simulink library "WECSim_Lib_Cables"  (R2020b)
settings: Solver=VariableStepAuto  StartTime=0.0  StopTime=10.0  RelTol=1e-3
undefined symbols (not defined in the file or in its folder): cable, simu, X, Y, Z
libraries: sm_lib x15, nesl_utility x13, vrlib x2, WECSim_Lib_Body_Elements x2
settings Model: Creator=kmruehl  LastModifiedBy=akeeste

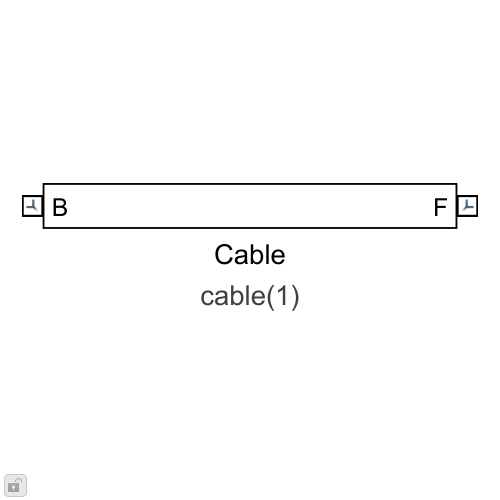
[thumbnail: Simulink's stored preview of the top-level diagram]
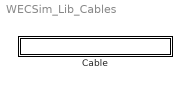
== system WECSim_Lib_Cables ==
  Cable : Subsystem  VariantControl=sv_Cable3DOF  mask(Cables){cable=cable(1)}
      mask prompts: cable "Cable Name:"
      mask help:
      | A cable that can be used to connect two bodies. If connecting a body to the seabed, use "Mooring" instead. This cable attaches to the body at either end with a spherical joint and applies damping and spring force between the bodies if the cable is in tension, and no force otherwise.
      |
      | The variable name input below must be 'cable(i)' where i=1,2,...
      | cable(i) must be defined in the input file with the following fields:
      |
      |   .name (required)
      | 	String.
      | 	Constraint name. Must comply with Matlab's variable naming rules.
      |   .stiffness (required)
      | 	The spring stiffness of the cable, applied externally as an actuation to the
      | 	translational PTO. This should be a strictly positive value for the cable to
      | 	act in tension. Default = 0
      |   .damping (required)
      | 	The damping coefficient of the cable, applied externally as an actuation to the
      | 	translational PTO. This should be a strictly positive value for the cable to
      | 	act in tension. Default = 0
      |   .length (optional)
      | 	The equilibrium length of the cable. If unspecified, it will be set at equilibrium
      | 	initially.
      |   .base.location (required)
      | 	The location of the top spherical joint connecting the cable to block base.
      | 	Default = [999 999 999]
      |   .follower.location (required)
      | 	The location of the bottom spherical joint connecting the cable to block follower.
      | 	Default = [999 999 999]
      mask init:
      | % toWorkspace
      | h=[gcb '/To Workspace'];
      | responseName=['cable' num2str((cable.number)) '_out'];
      | set_param(h,'VariableName',responseName);
      | 
      | %% follower drag body
      | % bodyMass constant
      | h=[gcb '/Follower Drag Body/Body Mass']; 
      | set_param(h,'Value', num2str(cable.mass));
      | % velocity GoTo
      | h=[gcb '/Follower Drag Body/Goto1'];
      | responseName=['cableVel' num2str((cable.number)) '_out1'];
      | set_param(h,'GotoTag',responseName);
      | % velocity From
      | h=[gcb '/Follower Drag Body/From1'];
      | responseName=['cableVel' num2str((cable.number)) '_out1'];
      | set_param(h,'GotoTag',responseName);
      | 
      | %% base drag body
      | % bodyMass constant
      | h=[gcb '/Base Drag Body/Body Mass']; 
      | set_param(h,'Value', num2str(cable.mass));
      | % velocity GoTo
      | h=[gcb '/Base Drag Body/Goto1'];
      | responseName=['cableVel' num2str((cable.number)) '_out2'];
      | set_param(h,'GotoTag',responseName);
      | % velocity From
      | h=[gcb '/Base Drag Body/From1'];
      | responseName=['cableVel' num2str((cable.number)) '_out2'];
      | set_param(h,'GotoTag',responseName);
      settings: AttributesFormatString=%<cable>
      mask Help:
      | A cable that can be used to connect two bodies. If connecting a body to the seabed, use "Mooring" instead. This cable attaches to the body at either end with a spherical joint and applies damping and spring force between the bodies if the cable is in tension, and no force otherwise.
      | 
      | The variable name input below must be 'cable(i)' where i=1,2,...
      | cable(i) must be defined in the input file with the following fields:
      | 
      |   .name (required)
      | 	String.
      | 	Constraint name. Must comply with Matlab's variable naming rules.
      |   .stiffness (required)
      | 	The spring stiffness of the cable, applied externally as an actuation to the
      | 	translational PTO. This should be a strictly positive value for the cable to
      | 	act in tension. Default = 0
      |   .damping (required)
      | 	The damping coefficient of the cable, applied externally as an actuation to the
      | 	translational PTO. This should be a strictly positive value for the cable to
      | 	act in tension. Default = 0
      |   .length (optional)
      | 	The equilibrium length of the cable. If unspecified, it will be set at equilibrium
      | 	initially.
      |   .base.location (required)
      | 	The location of the top spherical joint connecting the cable to block base.
      | 	Default = [999 999 999]
      |   .follower.location (required)
      | 	The location of the bottom spherical joint connecting the cable to block follower.
      | 	Default = [999 999 999]

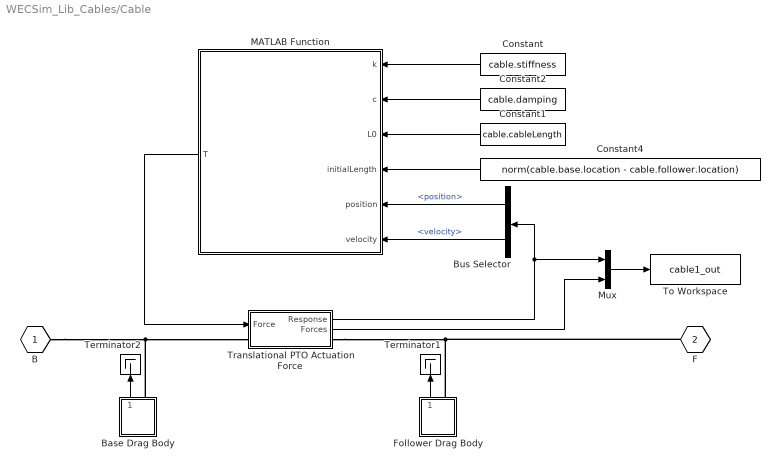
== system WECSim_Lib_Cables/Cable ==
  Base Drag Body : Subsystem  VariantControl=sv_b1_dragBody  mask(Drag Body){}
      mask help:
      | A drag body contains six degrees of freedom in x, y, z and Mx, My, Mz. It contains a buoyant force, linear damping force, and Morison Element and viscous forces. It is not influenced by wave excitation, radiation damping or radiation added mass.
      |
      | The variable name input below must be 'body(i)' where i=1,2,...
      | body(i) must be defined in the input file with the following fields:
      |
      |     .mass (required)
      |             Float or string.
      |             The translational interia or mass of the body in kg. If a string, the value must be 'equilibrium'. Default = [ ]
      |     .momOfIntertia (required)
      |             3x1 vector [Ixx Iyy Izz].
      |             Rotational intertia of the body in kg*m^2. Default = [ ]
      |     .filename (required)
      |             String.
      |             The file path specifying the .h5 file for the body.
      |     .name (optional)
      |             String.
      |             Specifies the body name. Default = [ ]
      |     .cg (optional)
      |             3x1 float vector [x y z]
      |     .cb (optional)
      |             3x1 float vector [x y z]
      |             Body center of buoyancy in m. Default = [ ].
      |     .volume (optional)
      |             Float.
      |             Displaced volume at the equilibrium position in m^3. Default = [ ]
      |     .geometryFile (optional)
      |             String
      |             Path to the geometry file of the body (.stl). Required for nonlinear hydrodynamics or visualization. Default = [ ]
  Bus Selector : BusSelector  OutputSignals=position,velocity
  Constant : Constant  Value=cable.stiffness
  Constant1 : Constant  Value=cable.cableLength
  Constant2 : Constant  Value=cable.damping
  Constant4 : Constant  Value=norm(cable.base.location - cable.follower.location)
  Follower Drag Body : Subsystem  VariantControl=sv_b1_dragBody  mask(Drag Body){}
      mask help:
      | A drag body contains six degrees of freedom in x, y, z and Mx, My, Mz. It contains a buoyant force, linear damping force, and Morison Element and viscous forces. It is not influenced by wave excitation, radiation damping or radiation added mass.
      |
      | The variable name input below must be 'body(i)' where i=1,2,...
      | body(i) must be defined in the input file with the following fields:
      |
      |     .mass (required)
      |             Float or string.
      |             The translational interia or mass of the body in kg. If a string, the value must be 'equilibrium'. Default = [ ]
      |     .momOfIntertia (required)
      |             3x1 vector [Ixx Iyy Izz].
      |             Rotational intertia of the body in kg*m^2. Default = [ ]
      |     .filename (required)
      |             String.
      |             The file path specifying the .h5 file for the body.
      |     .name (optional)
      |             String.
      |             Specifies the body name. Default = [ ]
      |     .cg (optional)
      |             3x1 float vector [x y z]
      |     .cb (optional)
      |             3x1 float vector [x y z]
      |             Body center of buoyancy in m. Default = [ ].
      |     .volume (optional)
      |             Float.
      |             Displaced volume at the equilibrium position in m^3. Default = [ ]
      |     .geometryFile (optional)
      |             String
      |             Path to the geometry file of the body (.stl). Required for nonlinear hydrodynamics or visualization. Default = [ ]
  MATLAB Function : MATLAB Function  TreatAsAtomicUnit=on
  Mux : Mux  Inputs=2
  Terminator1 : Terminator
  Terminator2 : Terminator
  To Workspace : ToWorkspace  VariableName=cable1_out  SaveFormat=Structure With Time  SampleTime=simu.dtOut
  Translational PTO Actuation Force : Subsystem  mask(PTO){cable=cable}
      mask help:
      | Constrains the follower to translational motion relative to the base, in
      | the PTO's Z-direction and adds PTO stiffness and damping. Also applies a
      | user-defined force and outputs extension, velocity, and acceleration.
      |
      |
      | The variable name input below must be 'pto(i)' where i=1,2,...
      | pto(i) must be defined in the input file with the following fields:
      |
      |     .name (required)
      |             String.
      |             PTO name. Must comply with Matlab's variable naming rules.
      |     .loc (optional)
      |             3x1 vector [x y z] in meters.
      |             PTO location. Default = [0 0 0]
      |     .k (optional)
      |             Float.
      |             PTO linear spring stiffness. Default = 0
      |     .c (optional)
      |             Float.
      |             PTO linear damping coefficient. Default = 0
      |     .orientation.z (optional)
      |             3x1 vector [x y z].
      |             Direction of the PTO's Z-coordinate. Default = [0 0 1]
      |     .orientation.y (optional)
      |             3x1 vector [x y z].
      |             Direction of the PTO's Y-coordinate. Default = [0 1 0]
      mask init:
      | cable.checkLoc('W');
      settings: AttributesFormatString=%<pto>
      mask Help:
      | Constraints the follower to translational motion relative to the base, in
      | the PTO's Z-direction and adds PTO stiffness and damping. Also applies a
      | user-defined force and outputs extension, velocity, and acceleration.
      | 
      | 
      | The variable name input below must be 'pto(i)' where i=1,2,...
      | pto(i) must be defined in the input file with the following fields:
      | 
      |     .name (required)
      |             String.
      |             PTO name. Must comply with Matlab's variable naming rules.
      |     .loc (optional)
      |             3x1 vector [x y z] in meters.
      |             PTO location. Default = [0 0 0]
      |     .k (optional)
      |             Float.
      |             PTO linear spring stiffness. Default = 0
      |     .c (optional)
      |             Float.
      |             PTO linear damping coefficient. Default = 0
      |     .orientation.z (optional)
      |             3x1 vector [x y z].
      |             Direction of the PTO's Z-coordinate. Default = [0 0 1]
      |     .orientation.y (optional)
      |             3x1 vector [x y z].
      |             Direction of the PTO's Y-coordinate. Default = [0 1 0]
  B : PMIOPort  Side=Left
  F : PMIOPort  Port=2  Side=Right
  wires:
  MATLAB Function/1(T) -> Translational PTO Actuation Force/1(Force)
  Translational PTO Actuation Force/1(Response) -> Mux/1, Bus Selector/1
  Mux/1 -> To Workspace/1
  Follower Drag Body/1(Output) -> Terminator1/1
  Base Drag Body/1(Output) -> Terminator2/1
  Constant1/1 -> MATLAB Function/3(L0)
  Constant/1 -> MATLAB Function/1(k)
  Constant2/1 -> MATLAB Function/2(c)
  Bus Selector/1 -> MATLAB Function/5(position)  "<position>"
  Bus Selector/2 -> MATLAB Function/6(velocity)  "<velocity>"
  Constant4/1 -> MATLAB Function/4(initialLength)
  Translational PTO Actuation Force/2("Forces ") -> Mux/2
  connections:
  Follower Drag Body/RConn1 -- F/RConn1 -- Translational PTO Actuation Force/RConn1
  B/RConn1 -- Base Drag Body/RConn1 -- Translational PTO Actuation Force/LConn1

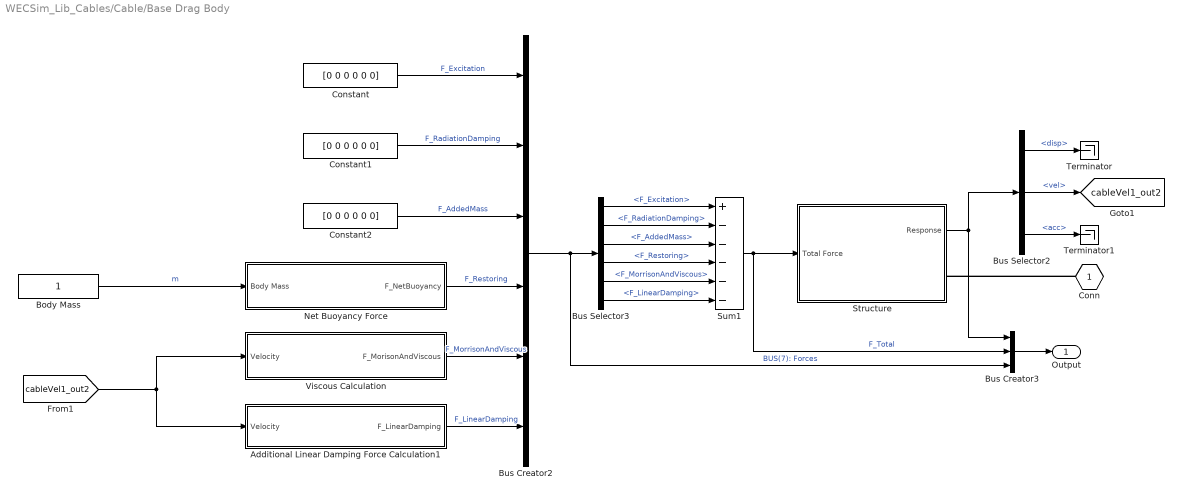
== system WECSim_Lib_Cables/Cable/Base Drag Body ==
  Additional Linear Damping Force Calculation1 : Subsystem
  Body Mass : Constant
  Bus Creator2 : BusCreator  Inputs=6
  Bus Creator3 : BusCreator  Inputs=3
  Bus Selector2 : BusSelector  OutputSignals=disp,vel,acc
  Bus Selector3 : BusSelector  OutputSignals=F_Excitation,F_RadiationDamping,F_AddedMass,F_Restoring,F_MorrisonAndViscous,F_LinearDamping
  Constant : Constant  Value=[0 0 0 0 0 0]
  Constant1 : Constant  Value=[0 0 0 0 0 0]
  Constant2 : Constant  Value=[0 0 0 0 0 0]
  Net Buoyancy Force : Subsystem
  Structure : Subsystem
  Sum1 : Sum  Inputs=+-----
  Terminator : Terminator
  Terminator1 : Terminator
  Viscous Calculation : Subsystem
  Conn : PMIOPort  Side=Right
  Output : Outport
  tag scope: cableVel1_out2=global
  wires:
  Body Mass/1 -> Net Buoyancy Force/1(Body Mass)  "m"
  [cableVel1_out2] -> Viscous Calculation/1(Velocity), Additional Linear Damping Force Calculation1/1(Velocity)
  Bus Selector3/6 -> Sum1/6  "<F_LinearDamping>"
  Bus Selector3/2 -> Sum1/2  "<F_RadiationDamping>"
  Constant2/1 -> Bus Creator2/3  "F_AddedMass"
  Sum1/1 -> Bus Creator3/2, Structure/1(Total Force)  "F_Total"
  Bus Creator2/1 -> Bus Creator3/3, Bus Selector3/1  "BUS(7): Forces"
  Bus Selector3/3 -> Sum1/3  "<F_AddedMass>"
  Bus Selector3/4 -> Sum1/4  "<F_Restoring>"
  Constant/1 -> Bus Creator2/1  "F_Excitation"
  Viscous Calculation/1(F_MorisonAndViscous) -> Bus Creator2/5  "F_MorrisonAndViscous"
  Additional Linear Damping Force Calculation1/1(F_LinearDamping) -> Bus Creator2/6  "F_LinearDamping"
  Net Buoyancy Force/1(F_NetBuoyancy) -> Bus Creator2/4  "F_Restoring"
  Bus Creator3/1 -> Output/1
  Constant1/1 -> Bus Creator2/2  "F_RadiationDamping"
  Bus Selector3/5 -> Sum1/5  "<F_MorrisonAndViscous>"
  Bus Selector3/1 -> Sum1/1  "<F_Excitation>"
  Bus Selector2/3 -> Terminator1/1  "<acc>"
  Bus Selector2/2 -> [cableVel1_out2]  "<vel>"
  Bus Selector2/1 -> Terminator/1  "<disp>"
  Structure/1(Response) -> Bus Selector2/1, Bus Creator3/1
  connections:
  Conn/RConn1 -- Structure/RConn1

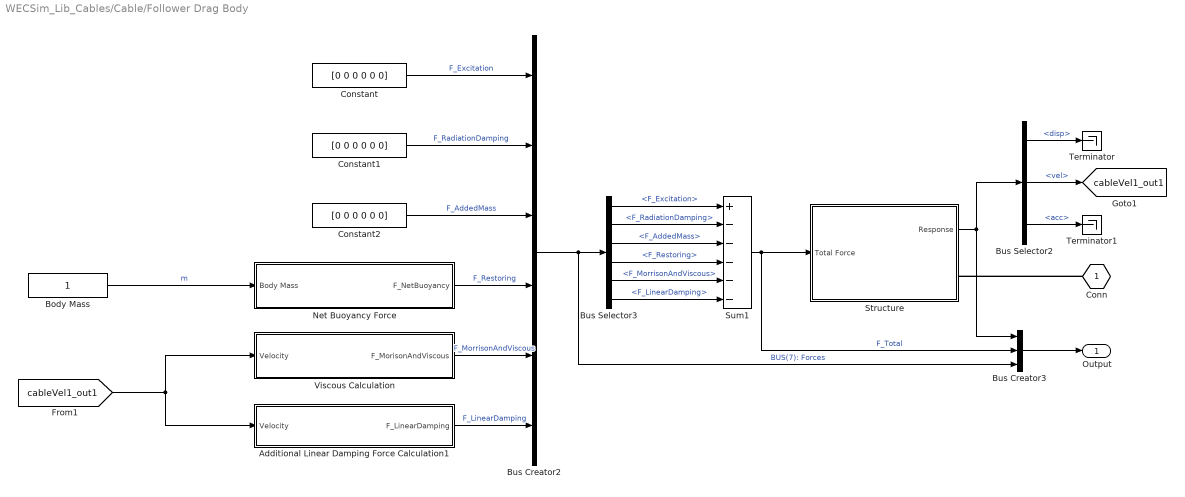
== system WECSim_Lib_Cables/Cable/Follower Drag Body ==
  Additional Linear Damping Force Calculation1 : Subsystem
  Body Mass : Constant
  Bus Creator2 : BusCreator  Inputs=6
  Bus Creator3 : BusCreator  Inputs=3
  Bus Selector2 : BusSelector  OutputSignals=disp,vel,acc
  Bus Selector3 : BusSelector  OutputSignals=F_Excitation,F_RadiationDamping,F_AddedMass,F_Restoring,F_MorrisonAndViscous,F_LinearDamping
  Constant : Constant  Value=[0 0 0 0 0 0]
  Constant1 : Constant  Value=[0 0 0 0 0 0]
  Constant2 : Constant  Value=[0 0 0 0 0 0]
  Net Buoyancy Force : Subsystem
  Structure : Subsystem
  Sum1 : Sum  Inputs=+-----
  Terminator : Terminator
  Terminator1 : Terminator
  Viscous Calculation : Subsystem
  Conn : PMIOPort  Side=Right
  Output : Outport
  tag scope: cableVel1_out1=global
  wires:
  Body Mass/1 -> Net Buoyancy Force/1(Body Mass)  "m"
  [cableVel1_out1] -> Additional Linear Damping Force Calculation1/1(Velocity), Viscous Calculation/1(Velocity)
  Bus Selector3/6 -> Sum1/6  "<F_LinearDamping>"
  Bus Selector3/2 -> Sum1/2  "<F_RadiationDamping>"
  Constant2/1 -> Bus Creator2/3  "F_AddedMass"
  Sum1/1 -> Bus Creator3/2, Structure/1(Total Force)  "F_Total"
  Bus Creator2/1 -> Bus Creator3/3, Bus Selector3/1  "BUS(7): Forces"
  Bus Selector3/3 -> Sum1/3  "<F_AddedMass>"
  Bus Selector3/4 -> Sum1/4  "<F_Restoring>"
  Constant/1 -> Bus Creator2/1  "F_Excitation"
  Viscous Calculation/1(F_MorisonAndViscous) -> Bus Creator2/5  "F_MorrisonAndViscous"
  Additional Linear Damping Force Calculation1/1(F_LinearDamping) -> Bus Creator2/6  "F_LinearDamping"
  Net Buoyancy Force/1(F_NetBuoyancy) -> Bus Creator2/4  "F_Restoring"
  Bus Creator3/1 -> Output/1
  Constant1/1 -> Bus Creator2/2  "F_RadiationDamping"
  Bus Selector3/5 -> Sum1/5  "<F_MorrisonAndViscous>"
  Bus Selector3/1 -> Sum1/1  "<F_Excitation>"
  Bus Selector2/1 -> Terminator/1  "<disp>"
  Bus Selector2/2 -> [cableVel1_out1]  "<vel>"
  Bus Selector2/3 -> Terminator1/1  "<acc>"
  Structure/1(Response) -> Bus Selector2/1, Bus Creator3/1
  connections:
  Conn/RConn1 -- Structure/RConn1

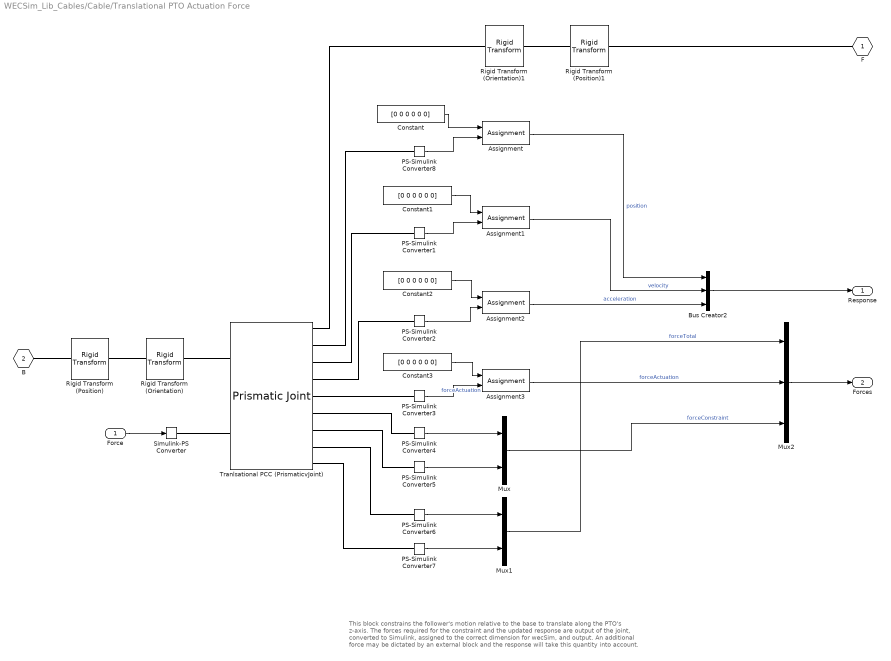
== system WECSim_Lib_Cables/Cable/Translational PTO Actuation Force ==
  note: This block constrains the follower's motion relative to the base to translate along the PTO's z-axis. The forces required for the constraint and the updated response are output of the joint, converted to Simulink, assigned to the correct dimension for wecSim, and output.
      |
      | An additional force may be dictated by an external block and the response will take this quantity into account.
  Force : Inport
  Assignment{,1..3} (4 alike) : Assignment  IndexOptions=Index vector (dialog)  Indices=3  OutputSizes=1
  Bus Creator2 : BusCreator  Inputs=3
  Constant{,1..3} (4 alike) : Constant  Value=[0 0 0 0 0 0]
  Mux : Mux  Inputs=2
  Mux1 : Mux  Inputs=2
  Mux2 : Mux  Inputs=3
  PS-Simulink Converter{1..8} (8 alike) : nesl_utility/PS-Simulink Converter  PhysicalDomain=network_engine_domain  SubClassName=ps_output  LeftPortType=input  RightPortType=output  PseudoPeriodic=off  Frequencies=[]  VectorFormat=1-D array  Unit=inherit  AffineConversion=off
  Rigid Transform (Position) : sm_lib/Frames and Transforms/Rigid Transform  RotationMethod=None  FollAlignAxisA=+X  BaseAlignAxisA=+Y  FollAlignAxisB=+Y  BaseAlignAxisB=+Z  RotationStandardAxis=+Z  RotationAngle=0.0  RotationAngleUnits=deg  RotationArbitraryAxis=[0 0 1]  RotationSequenceAxes=FollowerAxes  RotationSequence=XYX  RotationSequenceAngles=[0 0 0]  RotationSequenceAnglesUnits=deg  RotationMatrix=[1 0 0; 0 1 0; 0 0 1]  Quaternion=[1 0 0 0]  TranslationMethod=Cartesian  TranslationCartesianOffset=cable.initial.displacement+ cable.location  TranslationCartesianOffsetUnits=m  TranslationStandardAxis=+Z  TranslationStandardOffset=0  TranslationStandardOffsetUnits=m  TranslationROffset=0  TranslationROffsetUnits=m  TranslationThetaOffset=0  TranslationThetaOffsetUnits=deg  TranslationZOffset=0  TranslationZOffsetUnits=m
  Rigid Transform (Position)1 : sm_lib/Frames and Transforms/Rigid Transform  RotationMethod=None  FollAlignAxisA=+X  BaseAlignAxisA=+Y  FollAlignAxisB=+Y  BaseAlignAxisB=+Z  RotationStandardAxis=+Z  RotationAngle=0.0  RotationAngleUnits=deg  RotationArbitraryAxis=[0 0 1]  RotationSequenceAxes=FollowerAxes  RotationSequence=XYX  RotationSequenceAngles=[0 0 0]  RotationSequenceAnglesUnits=deg  RotationMatrix=[1 0 0; 0 1 0; 0 0 1]  Quaternion=[1 0 0 0]  TranslationMethod=Cartesian  TranslationCartesianOffset=cable.initial.displacement+ cable.location  TranslationCartesianOffsetUnits=m  TranslationStandardAxis=+Z  TranslationStandardOffset=0  TranslationStandardOffsetUnits=m  TranslationROffset=0  TranslationROffsetUnits=m  TranslationThetaOffset=0  TranslationThetaOffsetUnits=deg  TranslationZOffset=0  TranslationZOffsetUnits=m
  Rigid Transform (Orientation) : sm_lib/Frames and Transforms/Rigid Transform  RotationMethod=RotationMatrix  FollAlignAxisA=+X  BaseAlignAxisA=+Y  FollAlignAxisB=+Y  BaseAlignAxisB=+Z  RotationStandardAxis=+Z  RotationAngle=0.0  RotationAngleUnits=deg  RotationArbitraryAxis=[0 0 1]  RotationSequenceAxes=FollowerAxes  RotationSequence=XYX  RotationSequenceAngles=[0 0 0]  RotationSequenceAnglesUnits=deg  RotationMatrix=cable.orientation.rotationMatrix  Quaternion=[1 0 0 0]  TranslationMethod=None  TranslationCartesianOffset=cable.initial.displacement+ cable.location  TranslationCartesianOffsetUnits=m  TranslationStandardAxis=+Z  TranslationStandardOffset=0  TranslationStandardOffsetUnits=m  TranslationROffset=0  TranslationROffsetUnits=m  TranslationThetaOffset=0  TranslationThetaOffsetUnits=deg  TranslationZOffset=0  TranslationZOffsetUnits=m
  Rigid Transform (Orientation)1 : sm_lib/Frames and Transforms/Rigid Transform  RotationMethod=RotationMatrix  FollAlignAxisA=+X  BaseAlignAxisA=+Y  FollAlignAxisB=+Y  BaseAlignAxisB=+Z  RotationStandardAxis=+Z  RotationAngle=0.0  RotationAngleUnits=deg  RotationArbitraryAxis=[0 0 1]  RotationSequenceAxes=FollowerAxes  RotationSequence=XYX  RotationSequenceAngles=[0 0 0]  RotationSequenceAnglesUnits=deg  RotationMatrix=cable.orientation.rotationMatrix  Quaternion=[1 0 0 0]  TranslationMethod=None  TranslationCartesianOffset=cable.initial.displacement+ cable.location  TranslationCartesianOffsetUnits=m  TranslationStandardAxis=+Z  TranslationStandardOffset=0  TranslationStandardOffsetUnits=m  TranslationROffset=0  TranslationROffsetUnits=m  TranslationThetaOffset=0  TranslationThetaOffsetUnits=deg  TranslationZOffset=0  TranslationZOffsetUnits=m
  Simulink-PS Converter : nesl_utility/Simulink-PS Converter  PhysicalDomain=network_engine_domain  SubClassName=ps_input  LeftPortType=input  RightPortType=output  PseudoPeriodic=off  Frequencies=[]  NoiseDistribution=none  NoiseParameters=[]  Unit=1  AffineConversion=off  FilteringAndDerivatives=provide  SimscapeFilterOrder=1  InputFilterTimeConstant=0.001  UdotUserProvided=0
  Tranlsational PCC (PrismaticvJoint) : sm_lib/Joints/Prismatic Joint  JointMode=Normal  CompositeWrenchDir=BaseOnFollower  CompositeWrenchFrame=BaseFrame  SenseConstraintForce=on  SenseConstraintTorque=on  SenseTotalForce=on  SenseTotalTorque=on  PositionTargetSpecify=off  PositionTargetPriority=High  PositionTargetValue=0  PositionTargetValueUnits=m  VelocityTargetSpecify=off  VelocityTargetPriority=High  VelocityTargetValue=0  VelocityTargetValueUnits=m/s  EquilibriumPosition=0  EquilibriumPositionUnits=m  SpringStiffness=0  SpringStiffnessUnits=N/m  DampingCoefficient=0  DampingCoefficientUnits=N/(m/s)  LowerLimitSpecify=off  LowerLimitBound=-1  LowerLimitBoundUnits=m  LowerLimitStiffness=1e6  LowerLimitStiffnessUnits=N/m  LowerLimitDamping=1e3  LowerLimitDampingUnits=N/(m/s)  LowerLimitTransitionRegionWidth=1e-4  LowerLimitTransitionRegionWidthUnits=m  UpperLimitSpecify=off  UpperLimitBound=1  UpperLimitBoundUnits=m  UpperLimitStiffness=1e6  UpperLimitStiffnessUnits=N/m  UpperLimitDamping=1e3  UpperLimitDampingUnits=N/(m/s)  UpperLimitTransitionRegionWidth=1e-4  UpperLimitTransitionRegionWidthUnits=m  TorqueActuationMode=InputTorque  MotionActuationMode=ComputedMotion  SensePosition=on  SenseVelocity=on  SenseAcceleration=on  SenseTorqueForce=on  SenseLowerLimitTorqueForce=off  SenseUpperLimitTorqueForce=off
  F : PMIOPort  Side=Right
  B : PMIOPort  Port=2  Side=Left
  Response : Outport
  "Forces " : Outport  Port=2
  wires:
  PS-Simulink Converter3/1 -> Assignment3/2  "forceActuation"
  Constant3/1 -> Assignment3/1
  PS-Simulink Converter2/1 -> Assignment2/2
  Constant2/1 -> Assignment2/1
  PS-Simulink Converter1/1 -> Assignment1/2
  Constant1/1 -> Assignment1/1
  PS-Simulink Converter8/1 -> Assignment/2
  Constant/1 -> Assignment/1
  Assignment3/1 -> Mux2/2  "forceActuation"
  PS-Simulink Converter7/1 -> Mux1/2
  PS-Simulink Converter6/1 -> Mux1/1
  PS-Simulink Converter5/1 -> Mux/2
  PS-Simulink Converter4/1 -> Mux/1
  Mux1/1 -> Mux2/1  "forceTotal"
  Mux/1 -> Mux2/3  "forceConstraint"
  Mux2/1 -> "Forces "/1
  Force/1 -> Simulink-PS Converter/1
  Assignment2/1 -> Bus Creator2/3  "acceleration"
  Assignment1/1 -> Bus Creator2/2  "velocity"
  Assignment/1 -> Bus Creator2/1  "position"
  Bus Creator2/1 -> Response/1
  connections:
  Rigid Transform (Orientation)1/LConn1 -- Rigid Transform (Position)1/RConn1
  Rigid Transform (Position)/RConn1 -- Rigid Transform (Orientation)/LConn1
  PS-Simulink Converter4/LConn1 -- Tranlsational PCC (PrismaticvJoint)/RConn6
  PS-Simulink Converter8/LConn1 -- Tranlsational PCC (PrismaticvJoint)/RConn2
  PS-Simulink Converter6/LConn1 -- Tranlsational PCC (PrismaticvJoint)/RConn8
  Rigid Transform (Position)1/LConn1 -- F/RConn1
  PS-Simulink Converter1/LConn1 -- Tranlsational PCC (PrismaticvJoint)/RConn3
  PS-Simulink Converter5/LConn1 -- Tranlsational PCC (PrismaticvJoint)/RConn7
  PS-Simulink Converter2/LConn1 -- Tranlsational PCC (PrismaticvJoint)/RConn4
  Rigid Transform (Orientation)1/RConn1 -- Tranlsational PCC (PrismaticvJoint)/RConn1
  PS-Simulink Converter7/LConn1 -- Tranlsational PCC (PrismaticvJoint)/RConn9
  PS-Simulink Converter3/LConn1 -- Tranlsational PCC (PrismaticvJoint)/RConn5
  Rigid Transform (Position)/LConn1 -- B/RConn1
  Tranlsational PCC (PrismaticvJoint)/LConn1 -- Rigid Transform (Orientation)/RConn1
  Tranlsational PCC (PrismaticvJoint)/LConn2 -- Simulink-PS Converter/RConn1

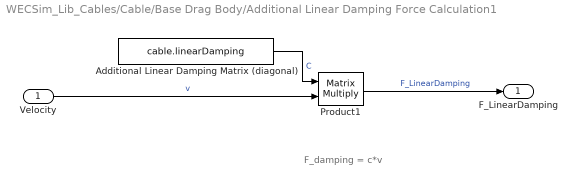
== system WECSim_Lib_Cables/Cable/Base Drag Body/Additional Linear Damping Force Calculation1 ==
  note: F_damping = c*v
  Velocity : Inport
  Additional Linear Damping Matrix (diagonal) : Constant  Value=cable.linearDamping
  Product1 : Product  Multiplication=Matrix(*)
  F_LinearDamping : Outport
  wires:
  Velocity/1 -> Product1/2  "v"
  Product1/1 -> F_LinearDamping/1  "F_LinearDamping"
  Additional Linear Damping Matrix (diagonal)/1 -> Product1/1  "C"

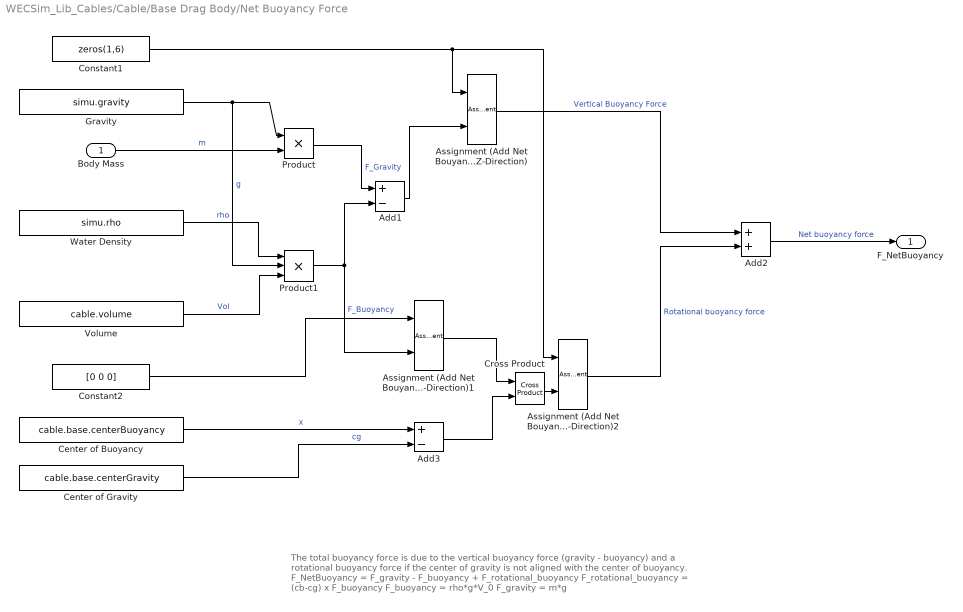
== system WECSim_Lib_Cables/Cable/Base Drag Body/Net Buoyancy Force ==
  note: The total buoyancy force is due to the vertical buoyancy force (gravity - buoyancy) and a rotational buoyancy force if the center of gravity is not aligned with the center of buoyancy.
      |
      | F_NetBuoyancy = F_gravity - F_buoyancy + F_rotational_buoyancy
      |
      | F_rotational_buoyancy = (cb-cg) x F_buoyancy
      | F_buoyancy = rho*g*V_0
      | F_gravity = m*g
  Body Mass : Inport
  Add1 : Sum  Inputs=+-
  Add2 : Sum
  Add3 : Sum  Inputs=+-
  Assignment (Add Net Bouyancy Force to Z-Direction) : Assignment  IndexOptions=Index vector (dialog)  Indices=3  OutputSizes=1
  Assignment (Add Net Bouyancy Force to Z-Direction)1 : Assignment  IndexOptions=Index vector (dialog)  Indices=3  OutputSizes=1
  Assignment (Add Net Bouyancy Force to Z-Direction)2 : Assignment  IndexOptions=Index vector (dialog)  Indices=4:6  OutputSizes=1
  Center of Buoyancy : Constant  Value=cable.base.centerBuoyancy
  Center of Gravity : Constant  Value=cable.base.centerGravity
  Constant1 : Constant  Value=zeros(1,6)
  Constant2 : Constant  Value=[0 0 0]
  Cross Product : vrlib/Utilities/Cross Product
  Gravity : Constant  Value=simu.gravity
  Product : Product
  Product1 : Product  Inputs=3
  Volume : Constant  Value=cable.volume
  Water Density : Constant  Value=simu.rho
  F_NetBuoyancy : Outport
  wires:
  Add1/1 -> Assignment (Add Net Bouyancy Force to Z-Direction)/2
  Body Mass/1 -> Product/2  "m"
  Cross Product/1 -> Assignment (Add Net Bouyancy Force to Z-Direction)2/2
  Add2/1 -> F_NetBuoyancy/1  "Net buoyancy force"
  Add3/1 -> Cross Product/2
  Constant2/1 -> Assignment (Add Net Bouyancy Force to Z-Direction)1/1
  Center of Gravity/1 -> Add3/2  "cg"
  Constant1/1 -> Assignment (Add Net Bouyancy Force to Z-Direction)/1, Assignment (Add Net Bouyancy Force to Z-Direction)2/1
  Center of Buoyancy/1 -> Add3/1  "x"
  Assignment (Add Net Bouyancy Force to Z-Direction)1/1 -> Cross Product/1
  Volume/1 -> Product1/3  "Vol"
  Assignment (Add Net Bouyancy Force to Z-Direction)/1 -> Add2/1  "Vertical Buoyancy Force"
  Water Density/1 -> Product1/1  "rho"
  Gravity/1 -> Product/1, Product1/2  "g"
  Product1/1 -> Assignment (Add Net Bouyancy Force to Z-Direction)1/2, Add1/2  "F_Buoyancy"
  Product/1 -> Add1/1  "F_Gravity"
  Assignment (Add Net Bouyancy Force to Z-Direction)2/1 -> Add2/2  "Rotational buoyancy force"

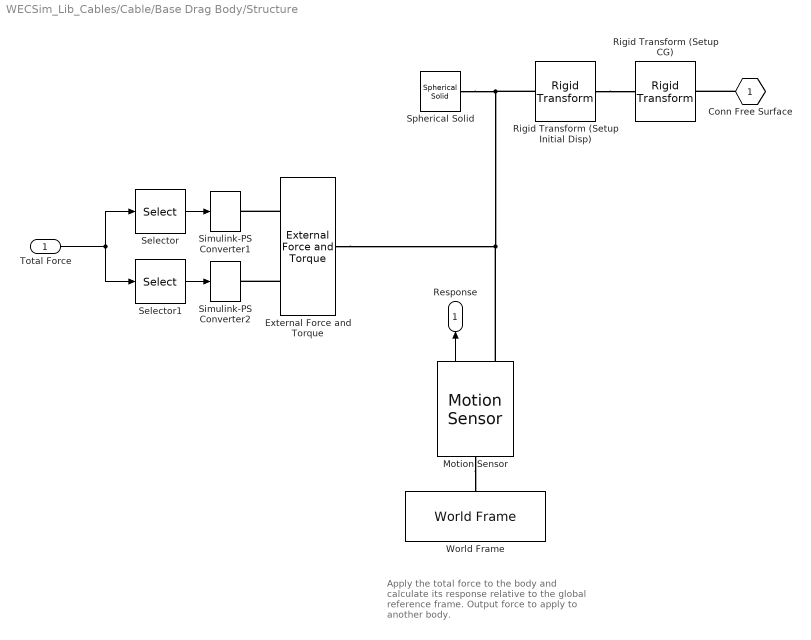
== system WECSim_Lib_Cables/Cable/Base Drag Body/Structure ==
  note: Apply the total force to the body and calculate its response relative to the global reference frame.
      |
      | Output force to apply to another body.
  Total Force : Inport
  External Force and Torque : sm_lib/Forces and Torques/External Force and Torque  EnableForceX=off  EnableForceY=off  EnableForceZ=off  EnableForce=on  ForceResolutionFrame=World  EnableTorqueX=off  EnableTorqueY=off  EnableTorqueZ=off  EnableTorque=on  TorqueResolutionFrame=World
  Motion Sensor : WECSim_Lib_Body_Elements/Rigid Body/Hydrodynamic Body/Structure/Motion Sensor  SystemSampleTime=-1  VariantActivationTime=update diagram  Latency=0  AutoFrameSizeCalculation=off
  Rigid Transform (Setup CG) : sm_lib/Frames and Transforms/Rigid Transform  RotationMethod=None  FollAlignAxisA=+X  BaseAlignAxisA=+Y  FollAlignAxisB=+Y  BaseAlignAxisB=+Z  RotationStandardAxis=+Y  RotationAngle=0.05  RotationAngleUnits=rad  RotationArbitraryAxis=[0.57735026918962584 0.57735026918962584 0.57735026918962584]  RotationSequenceAxes=FollowerAxes  RotationSequence=XYX  RotationSequenceAngles=[0 0 0]  RotationSequenceAnglesUnits=deg  RotationMatrix=[1 0 0; 0 1 0; 0 0 1]  Quaternion=[1 0 0 0]  TranslationMethod=Cartesian  TranslationCartesianOffset=cable.base.centerGravity  TranslationCartesianOffsetUnits=m  TranslationStandardAxis=+Z  TranslationStandardOffset=0  TranslationStandardOffsetUnits=m  TranslationROffset=0  TranslationROffsetUnits=m  TranslationThetaOffset=0  TranslationThetaOffsetUnits=deg  TranslationZOffset=0  TranslationZOffsetUnits=m
  Rigid Transform (Setup Initial Disp) : sm_lib/Frames and Transforms/Rigid Transform  RotationMethod=ArbitraryAxis  FollAlignAxisA=+X  BaseAlignAxisA=+Y  FollAlignAxisB=+Y  BaseAlignAxisB=+Z  RotationStandardAxis=+Y  RotationAngle=cable.initial.angle  RotationAngleUnits=rad  RotationArbitraryAxis=cable.initial.axis  RotationSequenceAxes=FollowerAxes  RotationSequence=XYX  RotationSequenceAngles=[0 0 0]  RotationSequenceAnglesUnits=deg  RotationMatrix=[1 0 0; 0 1 0; 0 0 1]  Quaternion=[1 0 0 0]  TranslationMethod=Cartesian  TranslationCartesianOffset=cable.initial.displacement  TranslationCartesianOffsetUnits=m  TranslationStandardAxis=+Z  TranslationStandardOffset=0  TranslationStandardOffsetUnits=m  TranslationROffset=0  TranslationROffsetUnits=m  TranslationThetaOffset=0  TranslationThetaOffsetUnits=deg  TranslationZOffset=0  TranslationZOffsetUnits=m
  Selector : Selector  InputPortWidth=6  IndexOptions=Index vector (dialog)  Indices=[1:3]  OutputSizes=1
  Selector1 : Selector  InputPortWidth=6  IndexOptions=Index vector (dialog)  Indices=[4:6]  OutputSizes=1
  Simulink-PS Converter1 : nesl_utility/Simulink-PS Converter  PhysicalDomain=network_engine_domain  SubClassName=ps_input  LeftPortType=input  RightPortType=output  PseudoPeriodic=off  Frequencies=[]  NoiseDistribution=none  NoiseParameters=[]  Unit=1  AffineConversion=off  FilteringAndDerivatives=zero  SimscapeFilterOrder=1  InputFilterTimeConstant=0.001  UdotUserProvided=1
  Simulink-PS Converter2 : nesl_utility/Simulink-PS Converter  PhysicalDomain=network_engine_domain  SubClassName=ps_input  LeftPortType=input  RightPortType=output  PseudoPeriodic=off  Frequencies=[]  NoiseDistribution=none  NoiseParameters=[]  Unit=1  AffineConversion=off  FilteringAndDerivatives=zero  SimscapeFilterOrder=1  InputFilterTimeConstant=0.001  UdotUserProvided=1
  Spherical Solid : sm_lib/Body Elements/Spherical Solid  SphereRadius=1  SphereRadiusUnits=m  ExportEntireGeometry=off  InertiaType=Custom  BasedOnType=Density  Density=1000  DensityUnits=kg/m^3  Mass=cable.mass  MassUnits=kg  CenterOfMass=[0 0 0]  CenterOfMassUnits=m  MomentsOfInertia=cable.inertia  MomentsOfInertiaUnits=kg*m^2  ProductsOfInertia=cable.inertiaProducts  ProductsOfInertiaUnits=kg*m^2  GraphicType=FromGeometry  MarkerShape=Sphere  MarkerSize=10  GraphicVisPropType=SimpleVisualProperties  GraphicDiffuseColor=[0.5 0.5 0.5]  GraphicOpacity=cable.viz.opacity  GraphicSpecularColor=[0.5 0.5 0.5 1.0]  GraphicAmbientColor=[0.15 0.15 0.15 1.0]  GraphicEmissiveColor=[0.0 0.0 0.0 1.0]  GraphicShininess=75  DoExposeReferenceFrame=on  SerializedFrames=<Frames/>
  World Frame : sm_lib/Frames and Transforms/World Frame
  Conn Free Surface : PMIOPort  Side=Right
  Response : Outport
  wires:
  Total Force/1 -> Selector1/1, Selector/1
  Selector/1 -> Simulink-PS Converter1/1
  Selector1/1 -> Simulink-PS Converter2/1
  Motion Sensor/1 -> Response/1
  connections:
  External Force and Torque/LConn1 -- Simulink-PS Converter1/RConn1
  External Force and Torque/LConn2 -- Simulink-PS Converter2/RConn1
  Rigid Transform (Setup Initial Disp)/RConn1 -- Spherical Solid/RConn1 -- Motion Sensor/RConn1 -- External Force and Torque/RConn1
  Conn Free Surface/RConn1 -- Rigid Transform (Setup CG)/LConn1
  Rigid Transform (Setup Initial Disp)/LConn1 -- Rigid Transform (Setup CG)/RConn1
  Motion Sensor/LConn1 -- World Frame/RConn1

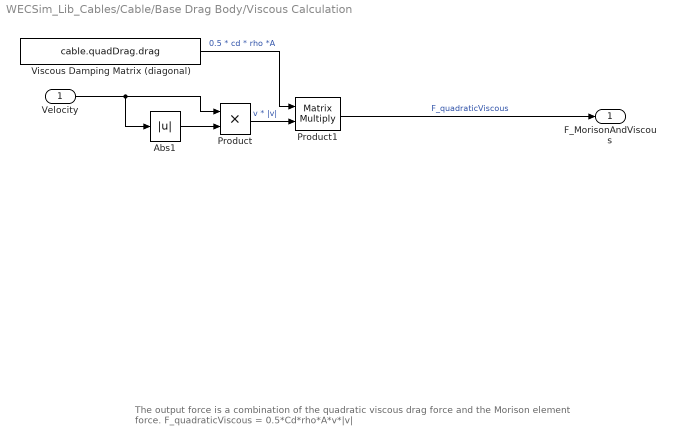
== system WECSim_Lib_Cables/Cable/Base Drag Body/Viscous Calculation ==
  note: The output force is a combination of the quadratic viscous drag force and the Morison element force.
      |
      | F_quadraticViscous = 0.5*Cd*rho*A*v*|v|
  Velocity : Inport
  Abs1 : Abs
  Product : Product
  Product1 : Product  Multiplication=Matrix(*)
  "Viscous Damping Matrix (diagonal) " : Constant  Value=cable.quadDrag.drag
  F_MorisonAndViscous : Outport
  wires:
  Velocity/1 -> Abs1/1, Product/1
  Product/1 -> Product1/2  "v * |v|"
  "Viscous Damping Matrix (diagonal) "/1 -> Product1/1  "0.5 * cd * rho *A"
  Product1/1 -> F_MorisonAndViscous/1  "F_quadraticViscous"
  Abs1/1 -> Product/2

== system WECSim_Lib_Cables/Cable/Follower Drag Body/Additional Linear Damping Force Calculation1 ==
  note: F_damping = c*v
  Velocity : Inport
  Additional Linear Damping Matrix (diagonal) : Constant  Value=cable.linearDamping
  Product1 : Product  Multiplication=Matrix(*)
  F_LinearDamping : Outport
  wires:
  Velocity/1 -> Product1/2  "v"
  Product1/1 -> F_LinearDamping/1  "F_LinearDamping"
  Additional Linear Damping Matrix (diagonal)/1 -> Product1/1  "C"

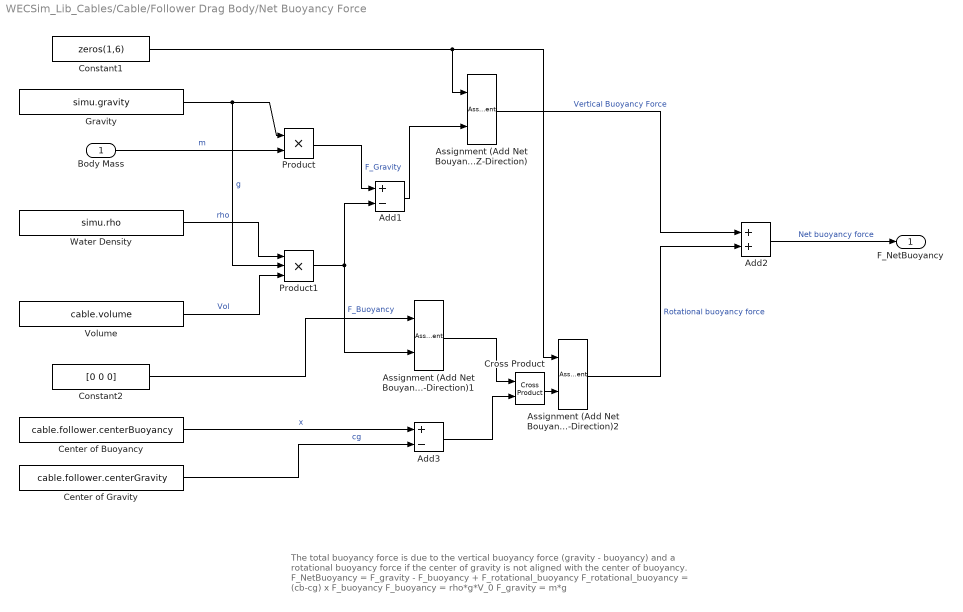
== system WECSim_Lib_Cables/Cable/Follower Drag Body/Net Buoyancy Force ==
  note: The total buoyancy force is due to the vertical buoyancy force (gravity - buoyancy) and a rotational buoyancy force if the center of gravity is not aligned with the center of buoyancy.
      |
      | F_NetBuoyancy = F_gravity - F_buoyancy + F_rotational_buoyancy
      |
      | F_rotational_buoyancy = (cb-cg) x F_buoyancy
      | F_buoyancy = rho*g*V_0
      | F_gravity = m*g
  Body Mass : Inport
  Add1 : Sum  Inputs=+-
  Add2 : Sum
  Add3 : Sum  Inputs=+-
  Assignment (Add Net Bouyancy Force to Z-Direction) : Assignment  IndexOptions=Index vector (dialog)  Indices=3  OutputSizes=1
  Assignment (Add Net Bouyancy Force to Z-Direction)1 : Assignment  IndexOptions=Index vector (dialog)  Indices=3  OutputSizes=1
  Assignment (Add Net Bouyancy Force to Z-Direction)2 : Assignment  IndexOptions=Index vector (dialog)  Indices=4:6  OutputSizes=1
  Center of Buoyancy : Constant  Value=cable.follower.centerBuoyancy
  Center of Gravity : Constant  Value=cable.follower.centerGravity
  Constant1 : Constant  Value=zeros(1,6)
  Constant2 : Constant  Value=[0 0 0]
  Cross Product : vrlib/Utilities/Cross Product
  Gravity : Constant  Value=simu.gravity
  Product : Product
  Product1 : Product  Inputs=3
  Volume : Constant  Value=cable.volume
  Water Density : Constant  Value=simu.rho
  F_NetBuoyancy : Outport
  wires:
  Add1/1 -> Assignment (Add Net Bouyancy Force to Z-Direction)/2
  Body Mass/1 -> Product/2  "m"
  Cross Product/1 -> Assignment (Add Net Bouyancy Force to Z-Direction)2/2
  Add2/1 -> F_NetBuoyancy/1  "Net buoyancy force"
  Add3/1 -> Cross Product/2
  Constant2/1 -> Assignment (Add Net Bouyancy Force to Z-Direction)1/1
  Center of Gravity/1 -> Add3/2  "cg"
  Constant1/1 -> Assignment (Add Net Bouyancy Force to Z-Direction)/1, Assignment (Add Net Bouyancy Force to Z-Direction)2/1
  Center of Buoyancy/1 -> Add3/1  "x"
  Assignment (Add Net Bouyancy Force to Z-Direction)1/1 -> Cross Product/1
  Volume/1 -> Product1/3  "Vol"
  Assignment (Add Net Bouyancy Force to Z-Direction)/1 -> Add2/1  "Vertical Buoyancy Force"
  Water Density/1 -> Product1/1  "rho"
  Gravity/1 -> Product/1, Product1/2  "g"
  Product1/1 -> Assignment (Add Net Bouyancy Force to Z-Direction)1/2, Add1/2  "F_Buoyancy"
  Product/1 -> Add1/1  "F_Gravity"
  Assignment (Add Net Bouyancy Force to Z-Direction)2/1 -> Add2/2  "Rotational buoyancy force"

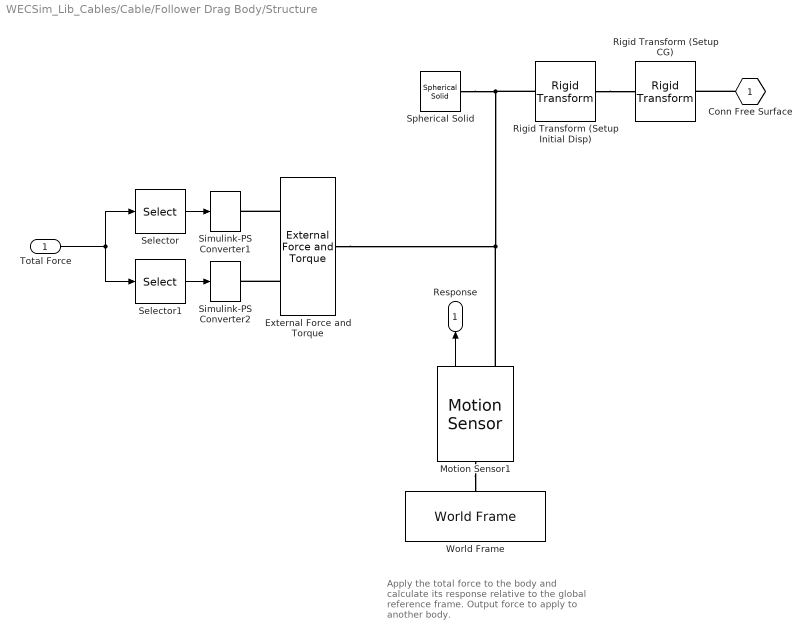
== system WECSim_Lib_Cables/Cable/Follower Drag Body/Structure ==
  note: Apply the total force to the body and calculate its response relative to the global reference frame.
      |
      | Output force to apply to another body.
  Total Force : Inport
  External Force and Torque : sm_lib/Forces and Torques/External Force and Torque  EnableForceX=off  EnableForceY=off  EnableForceZ=off  EnableForce=on  ForceResolutionFrame=World  EnableTorqueX=off  EnableTorqueY=off  EnableTorqueZ=off  EnableTorque=on  TorqueResolutionFrame=World
  Motion Sensor1 : WECSim_Lib_Body_Elements/Rigid Body/Hydrodynamic Body/Structure/Motion Sensor  SystemSampleTime=-1  VariantActivationTime=update diagram  Latency=0  AutoFrameSizeCalculation=off
  Rigid Transform (Setup CG) : sm_lib/Frames and Transforms/Rigid Transform  RotationMethod=None  FollAlignAxisA=+X  BaseAlignAxisA=+Y  FollAlignAxisB=+Y  BaseAlignAxisB=+Z  RotationStandardAxis=+Y  RotationAngle=0.05  RotationAngleUnits=rad  RotationArbitraryAxis=[0.57735026918962584 0.57735026918962584 0.57735026918962584]  RotationSequenceAxes=FollowerAxes  RotationSequence=XYX  RotationSequenceAngles=[0 0 0]  RotationSequenceAnglesUnits=deg  RotationMatrix=[1 0 0; 0 1 0; 0 0 1]  Quaternion=[1 0 0 0]  TranslationMethod=Cartesian  TranslationCartesianOffset=cable.follower.centerGravity  TranslationCartesianOffsetUnits=m  TranslationStandardAxis=+Z  TranslationStandardOffset=0  TranslationStandardOffsetUnits=m  TranslationROffset=0  TranslationROffsetUnits=m  TranslationThetaOffset=0  TranslationThetaOffsetUnits=deg  TranslationZOffset=0  TranslationZOffsetUnits=m
  Rigid Transform (Setup Initial Disp) : sm_lib/Frames and Transforms/Rigid Transform  RotationMethod=ArbitraryAxis  FollAlignAxisA=+X  BaseAlignAxisA=+Y  FollAlignAxisB=+Y  BaseAlignAxisB=+Z  RotationStandardAxis=+Y  RotationAngle=cable.initial.angle  RotationAngleUnits=rad  RotationArbitraryAxis=cable.initial.axis  RotationSequenceAxes=FollowerAxes  RotationSequence=XYX  RotationSequenceAngles=[0 0 0]  RotationSequenceAnglesUnits=deg  RotationMatrix=[1 0 0; 0 1 0; 0 0 1]  Quaternion=[1 0 0 0]  TranslationMethod=Cartesian  TranslationCartesianOffset=cable.initial.displacement  TranslationCartesianOffsetUnits=m  TranslationStandardAxis=+Z  TranslationStandardOffset=0  TranslationStandardOffsetUnits=m  TranslationROffset=0  TranslationROffsetUnits=m  TranslationThetaOffset=0  TranslationThetaOffsetUnits=deg  TranslationZOffset=0  TranslationZOffsetUnits=m
  Selector : Selector  InputPortWidth=6  IndexOptions=Index vector (dialog)  Indices=[1:3]  OutputSizes=1
  Selector1 : Selector  InputPortWidth=6  IndexOptions=Index vector (dialog)  Indices=[4:6]  OutputSizes=1
  Simulink-PS Converter1 : nesl_utility/Simulink-PS Converter  PhysicalDomain=network_engine_domain  SubClassName=ps_input  LeftPortType=input  RightPortType=output  PseudoPeriodic=off  Frequencies=[]  NoiseDistribution=none  NoiseParameters=[]  Unit=1  AffineConversion=off  FilteringAndDerivatives=zero  SimscapeFilterOrder=1  InputFilterTimeConstant=0.001  UdotUserProvided=1
  Simulink-PS Converter2 : nesl_utility/Simulink-PS Converter  PhysicalDomain=network_engine_domain  SubClassName=ps_input  LeftPortType=input  RightPortType=output  PseudoPeriodic=off  Frequencies=[]  NoiseDistribution=none  NoiseParameters=[]  Unit=1  AffineConversion=off  FilteringAndDerivatives=zero  SimscapeFilterOrder=1  InputFilterTimeConstant=0.001  UdotUserProvided=1
  Spherical Solid : sm_lib/Body Elements/Spherical Solid  SphereRadius=1  SphereRadiusUnits=m  ExportEntireGeometry=off  InertiaType=Custom  BasedOnType=Density  Density=1000  DensityUnits=kg/m^3  Mass=cable.mass  MassUnits=kg  CenterOfMass=[0 0 0]  CenterOfMassUnits=m  MomentsOfInertia=cable.inertia  MomentsOfInertiaUnits=kg*m^2  ProductsOfInertia=cable.inertiaProducts  ProductsOfInertiaUnits=kg*m^2  GraphicType=FromGeometry  MarkerShape=Sphere  MarkerSize=10  GraphicVisPropType=SimpleVisualProperties  GraphicDiffuseColor=[0.5 0.5 0.5]  GraphicOpacity=cable.viz.opacity  GraphicSpecularColor=[0.5 0.5 0.5 1.0]  GraphicAmbientColor=[0.15 0.15 0.15 1.0]  GraphicEmissiveColor=[0.0 0.0 0.0 1.0]  GraphicShininess=75  DoExposeReferenceFrame=on  SerializedFrames=<Frames/>
  World Frame : sm_lib/Frames and Transforms/World Frame
  Conn Free Surface : PMIOPort  Side=Right
  Response : Outport
  wires:
  Total Force/1 -> Selector1/1, Selector/1
  Selector/1 -> Simulink-PS Converter1/1
  Selector1/1 -> Simulink-PS Converter2/1
  Motion Sensor1/1 -> Response/1
  connections:
  External Force and Torque/LConn1 -- Simulink-PS Converter1/RConn1
  External Force and Torque/LConn2 -- Simulink-PS Converter2/RConn1
  Rigid Transform (Setup Initial Disp)/RConn1 -- Spherical Solid/RConn1 -- Motion Sensor1/RConn1 -- External Force and Torque/RConn1
  Conn Free Surface/RConn1 -- Rigid Transform (Setup CG)/LConn1
  Rigid Transform (Setup Initial Disp)/LConn1 -- Rigid Transform (Setup CG)/RConn1
  Motion Sensor1/LConn1 -- World Frame/RConn1

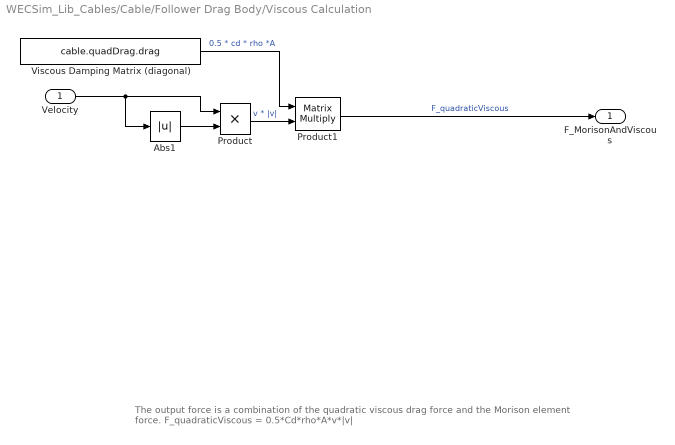
== system WECSim_Lib_Cables/Cable/Follower Drag Body/Viscous Calculation ==
  note: The output force is a combination of the quadratic viscous drag force and the Morison element force.
      |
      | F_quadraticViscous = 0.5*Cd*rho*A*v*|v|
  Velocity : Inport
  Abs1 : Abs
  Product : Product
  Product1 : Product  Multiplication=Matrix(*)
  "Viscous Damping Matrix (diagonal) " : Constant  Value=cable.quadDrag.drag
  F_MorisonAndViscous : Outport
  wires:
  Velocity/1 -> Abs1/1, Product/1
  Product/1 -> Product1/2  "v * |v|"
  "Viscous Damping Matrix (diagonal) "/1 -> Product1/1  "0.5 * cd * rho *A"
  Product1/1 -> F_MorisonAndViscous/1  "F_quadraticViscous"
  Abs1/1 -> Product/2

== matlab function WECSim_Lib_Cables/Cable/MATLAB Function ==
  data: k input; c input; L0 input; initialLength input; position input; T output; velocity input
function T = calcCableTens(k, c, L0, initialLength, position, velocity)

T = calcCableTens(k, c, L0, initialLength, position, velocity);

end
